simulink model "pid_saturation_simulink"  (R2022b)
settings: Solver=ode45  StartTime=0.0  StopTime=30  MaxStep=0.005  RelTol=1e-8  AbsTol=1e-10
settings Model: Creator=邵  LastModifiedBy=邵

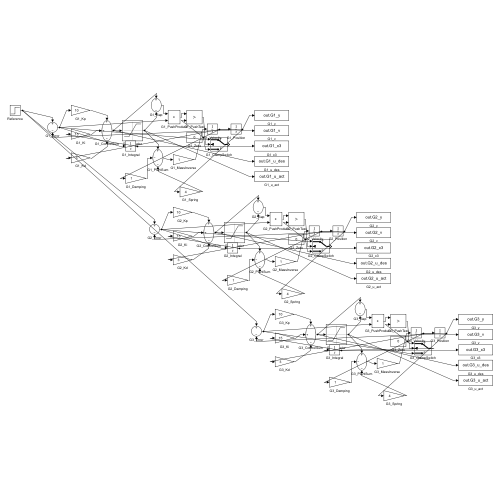
[thumbnail: Simulink's stored preview of the top-level diagram]
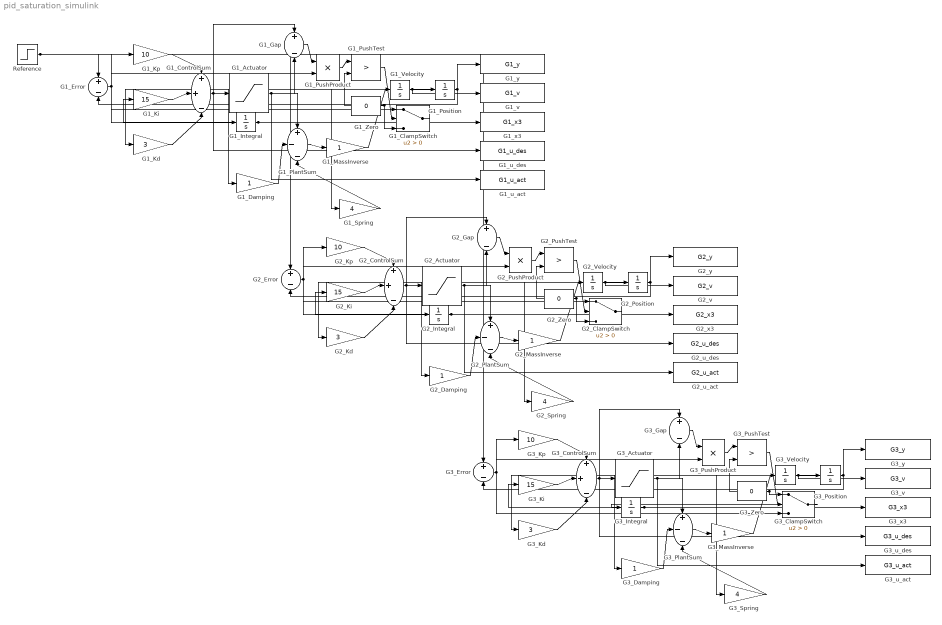
== system pid_saturation_simulink ==
  G1_Actuator : Saturate  UpperLimit=Inf  LowerLimit=-Inf
  G1_ClampSwitch : Switch  Criteria=u2 > Threshold  SaturateOnIntegerOverflow=off  InputSameDT=off
  G1_ControlSum : Sum  Inputs=++-
  G1_Damping : Gain
  G1_Error : Sum  Inputs=+-
  G1_Gap : Sum  Inputs=+-
  G1_Integral : Integrator
  G1_Kd : Gain  Gain=3
  G1_Ki : Gain  Gain=15
  G1_Kp : Gain  Gain=10
  G1_MassInverse : Gain
  G1_PlantSum : Sum  Inputs=+--
  G1_Position : Integrator
  G1_PushProduct : Product
  G1_PushTest : RelationalOperator  Operator=>  OutDataTypeStr=boolean  RndMeth=Simplest  InputSameDT=off
  G1_Spring : Gain  Gain=4
  G1_Velocity : Integrator
  G1_Zero : Constant  Value=0
  G1_u_act : ToWorkspace  VariableName=G1_u_act  SaveFormat=Structure With Time  SampleTime=-1
  G1_u_des : ToWorkspace  VariableName=G1_u_des  SaveFormat=Structure With Time  SampleTime=-1
  G1_v : ToWorkspace  VariableName=G1_v  SaveFormat=Structure With Time  SampleTime=-1
  G1_x3 : ToWorkspace  VariableName=G1_x3  SaveFormat=Structure With Time  SampleTime=-1
  G1_y : ToWorkspace  VariableName=G1_y  SaveFormat=Structure With Time  SampleTime=-1
  G2_Actuator : Saturate  UpperLimit=5  LowerLimit=-5
  G2_ClampSwitch : Switch  Criteria=u2 > Threshold  SaturateOnIntegerOverflow=off  InputSameDT=off
  G2_ControlSum : Sum  Inputs=++-
  G2_Damping : Gain
  G2_Error : Sum  Inputs=+-
  G2_Gap : Sum  Inputs=+-
  G2_Integral : Integrator
  G2_Kd : Gain  Gain=3
  G2_Ki : Gain  Gain=15
  G2_Kp : Gain  Gain=10
  G2_MassInverse : Gain
  G2_PlantSum : Sum  Inputs=+--
  G2_Position : Integrator
  G2_PushProduct : Product
  G2_PushTest : RelationalOperator  Operator=>  OutDataTypeStr=boolean  RndMeth=Simplest  InputSameDT=off
  G2_Spring : Gain  Gain=4
  G2_Velocity : Integrator
  G2_Zero : Constant  Value=0
  G2_u_act : ToWorkspace  VariableName=G2_u_act  SaveFormat=Structure With Time  SampleTime=-1
  G2_u_des : ToWorkspace  VariableName=G2_u_des  SaveFormat=Structure With Time  SampleTime=-1
  G2_v : ToWorkspace  VariableName=G2_v  SaveFormat=Structure With Time  SampleTime=-1
  G2_x3 : ToWorkspace  VariableName=G2_x3  SaveFormat=Structure With Time  SampleTime=-1
  G2_y : ToWorkspace  VariableName=G2_y  SaveFormat=Structure With Time  SampleTime=-1
  G3_Actuator : Saturate  UpperLimit=5  LowerLimit=-5
  G3_ClampSwitch : Switch  Criteria=u2 > Threshold  SaturateOnIntegerOverflow=off  InputSameDT=off
  G3_ControlSum : Sum  Inputs=++-
  G3_Damping : Gain
  G3_Error : Sum  Inputs=+-
  G3_Gap : Sum  Inputs=+-
  G3_Integral : Integrator
  G3_Kd : Gain  Gain=3
  G3_Ki : Gain  Gain=15
  G3_Kp : Gain  Gain=10
  G3_MassInverse : Gain
  G3_PlantSum : Sum  Inputs=+--
  G3_Position : Integrator
  G3_PushProduct : Product
  G3_PushTest : RelationalOperator  Operator=>  OutDataTypeStr=boolean  RndMeth=Simplest  InputSameDT=off
  G3_Spring : Gain  Gain=4
  G3_Velocity : Integrator
  G3_Zero : Constant  Value=0
  G3_u_act : ToWorkspace  VariableName=G3_u_act  SaveFormat=Structure With Time  SampleTime=-1
  G3_u_des : ToWorkspace  VariableName=G3_u_des  SaveFormat=Structure With Time  SampleTime=-1
  G3_v : ToWorkspace  VariableName=G3_v  SaveFormat=Structure With Time  SampleTime=-1
  G3_x3 : ToWorkspace  VariableName=G3_x3  SaveFormat=Structure With Time  SampleTime=-1
  G3_y : ToWorkspace  VariableName=G3_y  SaveFormat=Structure With Time  SampleTime=-1
  Reference : Step  Time=0  SampleTime=0
  wires:
  Reference/1 -> G1_Error/1, G2_Error/1, G3_Error/1
  G1_Position/1 -> G1_Error/2, G1_Spring/1, G1_y/1
  G1_Error/1 -> G1_Kp/1, G1_PushProduct/2, G1_ClampSwitch/1, G1_Integral/1
  G1_Velocity/1 -> G1_Kd/1, G1_Damping/1, G1_Position/1, G1_v/1
  G1_Kp/1 -> G1_ControlSum/1
  G1_Ki/1 -> G1_ControlSum/2
  G1_Kd/1 -> G1_ControlSum/3
  G1_ControlSum/1 -> G1_Actuator/1, G1_Gap/1, G1_u_des/1
  G1_Actuator/1 -> G1_Gap/2, G1_PlantSum/1, G1_u_act/1
  G1_Gap/1 -> G1_PushProduct/1
  G1_PushProduct/1 -> G1_PushTest/1
  G1_Zero/1 -> G1_PushTest/2, G1_ClampSwitch/3
  G1_PushTest/1 -> G1_ClampSwitch/2
  G1_Damping/1 -> G1_PlantSum/2
  G1_Spring/1 -> G1_PlantSum/3
  G1_PlantSum/1 -> G1_MassInverse/1
  G1_MassInverse/1 -> G1_Velocity/1
  G1_Integral/1 -> G1_x3/1, G1_Ki/1
  G2_Position/1 -> G2_Error/2, G2_Spring/1, G2_y/1
  G2_Error/1 -> G2_Kp/1, G2_PushProduct/2, G2_ClampSwitch/1, G2_Integral/1
  G2_Velocity/1 -> G2_Kd/1, G2_Damping/1, G2_Position/1, G2_v/1
  G2_Kp/1 -> G2_ControlSum/1
  G2_Ki/1 -> G2_ControlSum/2
  G2_Kd/1 -> G2_ControlSum/3
  G2_ControlSum/1 -> G2_Actuator/1, G2_Gap/1, G2_u_des/1
  G2_Actuator/1 -> G2_Gap/2, G2_PlantSum/1, G2_u_act/1
  G2_Gap/1 -> G2_PushProduct/1
  G2_PushProduct/1 -> G2_PushTest/1
  G2_Zero/1 -> G2_PushTest/2, G2_ClampSwitch/3
  G2_PushTest/1 -> G2_ClampSwitch/2
  G2_Damping/1 -> G2_PlantSum/2
  G2_Spring/1 -> G2_PlantSum/3
  G2_PlantSum/1 -> G2_MassInverse/1
  G2_MassInverse/1 -> G2_Velocity/1
  G2_Integral/1 -> G2_x3/1, G2_Ki/1
  G3_Position/1 -> G3_Error/2, G3_Spring/1, G3_y/1
  G3_Error/1 -> G3_Kp/1, G3_PushProduct/2, G3_ClampSwitch/3
  G3_Velocity/1 -> G3_Kd/1, G3_Damping/1, G3_Position/1, G3_v/1
  G3_Kp/1 -> G3_ControlSum/1
  G3_Ki/1 -> G3_ControlSum/2
  G3_Kd/1 -> G3_ControlSum/3
  G3_ControlSum/1 -> G3_Actuator/1, G3_Gap/1, G3_u_des/1
  G3_Actuator/1 -> G3_Gap/2, G3_PlantSum/1, G3_u_act/1
  G3_Gap/1 -> G3_PushProduct/1
  G3_PushProduct/1 -> G3_PushTest/1
  G3_Zero/1 -> G3_PushTest/2, G3_ClampSwitch/1
  G3_PushTest/1 -> G3_ClampSwitch/2
  G3_ClampSwitch/1 -> G3_Integral/1
  G3_Damping/1 -> G3_PlantSum/2
  G3_Spring/1 -> G3_PlantSum/3
  G3_PlantSum/1 -> G3_MassInverse/1
  G3_MassInverse/1 -> G3_Velocity/1
  G3_Integral/1 -> G3_x3/1, G3_Ki/1
